simulink model "EMT_ML"  (R2024b)
settings: Solver=ode5  StartTime=0.0  StopTime=200  FixedStep=0.002  RelTol=1e-3
model workspace (MAT data in the model file):
  A = 7.3
  B = 2.71
  C0_shift = 200
  C1_shift = 200
  C2_shift = 200
  Cb = 70
  Cd = 0.6
  EMSInputBus = Simulink.Bus
  EMSInputBus.Alignment = -1
  EMSInputBus.PreserveElementDimensions = 0
  EMSInputBus.Elements_internal(1) = Simulink.BusElement
  EMSInputBus.Elements_internal(1).DimensionsMode = 'Fixed'
  EMSInputBus.Elements_internal(1).SamplingMode = 'Sample based'
  EMSInputBus.Elements_internal(1).SampleTime = -1
  EMSInputBus.Elements_internal(1).Name = 'legacy'
  EMSInputBus.Elements_internal(1).DataType_internal = 'double'
  EMSInputBus.Elements_internal(1).Complexity = 'real'
  EMSInputBus.Elements_internal(1).Dimensions = 19
  EMSInputBus.Elements_internal(2) = Simulink.BusElement
  EMSInputBus.Elements_internal(2).DimensionsMode = 'Fixed'
  EMSInputBus.Elements_internal(2).SamplingMode = 'Sample based'
  EMSInputBus.Elements_internal(2).SampleTime = -1
  EMSInputBus.Elements_internal(2).Name = 'observation'
  EMSInputBus.Elements_internal(2).DataType_internal = 'double'
  EMSInputBus.Elements_internal(2).Complexity = 'real'
  EMSInputBus.Elements_internal(2).Dimensions = 20
  EMSInputBus.Elements_internal(3) = Simulink.BusElement
  EMSInputBus.Elements_internal(3).DimensionsMode = 'Fixed'
  EMSInputBus.Elements_internal(3).SamplingMode = 'Sample based'
  EMSInputBus.Elements_internal(3).SampleTime = -1
  EMSInputBus.Elements_internal(3).Name = 'original_action'
  EMSInputBus.Elements_internal(3).DataType_internal = 'double'
  EMSInputBus.Elements_internal(3).Complexity = 'real'
  EMSInputBus.Elements_internal(3).Dimensions = 4
  EMSInputBus.DataScope = 'Auto'
  Fb_max = 247500
  JA = 0.4
  JB = 0.4
  JZ = 0.4
  Jc1r2 = 0.01
  Jc3r4 = 0.01
  Jc4 = 0.01
  Je = 2.5
  Jh = 0.01
  Jq1 = 0.01
  Jq2 = 0.01
  Jr1 = 0.01
  Jr3s4 = 0.01
  Js123 = 0.01
  L = 4.472
  NE = [1600 1600 1600 1600 1600 1600 1600 1600 1600 1600 1600 1600 ... (840 elements, 30x28)]
  N_Te = 30
  N_ne = 28
  PE = [0 100.366530527 133.710336161 167.221698607 195.706356687 221.845219395 250.497434286 278.144308305 305.288511886 330.086920096 352.87464656 374.489475338 ... (840 elements, 30x28)]
  PN0 = 0
  Pb_epr = [-45 -45 -40 -30 0 30 40 45 45]
  Pb_max = [0 40 45 45 45]
  Pb_min = [-45 -45 -45 -40 0]
  Pe_ass = 230
  Pe_max = 1103
  Peg = [0 100 120 140 160 180 200 220 240 260 280 300 320 340 360 380 400 420 440 460 480 500 520 540 560 580 600 620 640 660 680 700 720 740 760 780 800 820 840 860 880 900 920 940 960 980 1000 1020 1040 1060 1080 1100 1200]
  R_map = [0.09 0.089 0.09 0.091 0.092 0.093 0.094 0.095 0.096 0.097 0.098]
  SF_C0 = 1.5
  SF_C1 = 1.5
  SF_C2 = 1.5
  SF_Z1 = 1.5
  SF_Z2 = 1.5
  SF_ZD = 1.5
  SOC0 = 60
  SOC_epr = [30 31 50 59 60 61 70 79 80]
  SOC_map = [0 10 20 30 40 50 60 70 80 90 100]
  TA_max_map = [588.855 593.803361345 598.83559322 603.953846154 609.160344828 614.457391304 619.847368421 625.332743363 630.916071429 636.6 642.387272727 648.280733945 654.283333333 660.398130841 666.628301887 672.977142857 679.448076923 686.044660194 692.770588235 699.62970297 706.626 713.763636364 721.046938776 728.480412371 736.06875 743.816842105 751.729787234 759.812903226 768.07173913 776.512087912 785.14 793.961797753 802.984090909 812.213793103 821.658139535 831.324705882 841.221428571 851.356626506 861.73902439 872.377777778 883.2825 894.463291139 905.930769231 917.696103896 929.771052632 942.168 954.9 967.980821918 981.425 995.247887324 1009.46571429 1024.09565217 1039.15588235 1054.66567164 1070.64545455 1087.11692308 1110 1110 1110 1087.11692308 1070.64545455 1054.66567164 1039.15588235 1024.09565217 1009.46571429 995.247887324 981.425 967.980821918 954.9 942.168 929.771052632 917.696103896 905.930769231 894.463291139 883.2825 872.377777778 861.73902439 851.356626506 841.221428571 831.324705882 821.658139535 812.213793103 802.984090909 793.961797753 785.14 776.512087912 768.07173913 759.812903226 751.729787234 743.816842105 736.06875 728.480412371 721.046938776 713.763636364 706.626 699.62970297 692.770588235 686.044660194 679.448076923 672.977142857 666.628301887 660.398130841 654.283333333 648.280733945 642.387272727 636.6 630.916071429 625.332743363 619.847368421 614.457391304 609.160344828 603.953846154 598.83559322 593.803361345 588.855]
  TA_min_map = [-588.855 -593.803361345 -598.83559322 -603.953846154 -609.160344828 -614.457391304 -619.847368421 -625.332743363 -630.916071429 -636.6 -642.387272727 -648.280733945 -654.283333333 -660.398130841 -666.628301887 -672.977142857 -679.448076923 -686.044660194 -692.770588235 -699.62970297 -706.626 -713.763636364 -721.046938776 -728.480412371 -736.06875 -743.816842105 -751.729787234 -759.812903226 -768.07173913 -776.512087912 -785.14 -793.961797753 -802.984090909 -812.213793103 -821.658139535 -831.324705882 -841.221428571 -851.356626506 -861.73902439 -872.377777778 -883.2825 -894.463291139 -905.930769231 -917.696103896 -929.771052632 -942.168 -954.9 -967.980821918 -981.425 -995.247887324 -1009.46571429 -1024.09565217 -1039.15588235 -1054.66567164 -1070.64545455 -1087.11692308 -1110 -1110 -1110 -1087.11692308 -1070.64545455 -1054.66567164 -1039.15588235 -1024.09565217 -1009.46571429 -995.247887324 -981.425 -967.980821918 -954.9 -942.168 -929.771052632 -917.696103896 -905.930769231 -894.463291139 -883.2825 -872.377777778 -861.73902439 -851.356626506 -841.221428571 -831.324705882 -821.658139535 -812.213793103 -802.984090909 -793.961797753 -785.14 -776.512087912 -768.07173913 -759.812903226 -751.729787234 -743.816842105 -736.06875 -728.480412371 -721.046938776 -713.763636364 -706.626 -699.62970297 -692.770588235 -686.044660194 -679.448076923 -672.977142857 -666.628301887 -660.398130841 -654.283333333 -648.280733945 -642.387272727 -636.6 -630.916071429 -625.332743363 -619.847368421 -614.457391304 -609.160344828 -603.953846154 -598.83559322 -593.803361345 -588.855]
  TAf = 0
  TB_max_map = [588.855 593.803361345 598.83559322 603.953846154 609.160344828 614.457391304 619.847368421 625.332743363 630.916071429 636.6 642.387272727 648.280733945 654.283333333 660.398130841 666.628301887 672.977142857 679.448076923 686.044660194 692.770588235 699.62970297 706.626 713.763636364 721.046938776 728.480412371 736.06875 743.816842105 751.729787234 759.812903226 768.07173913 776.512087912 785.14 793.961797753 802.984090909 812.213793103 821.658139535 831.324705882 841.221428571 851.356626506 861.73902439 872.377777778 883.2825 894.463291139 905.930769231 917.696103896 929.771052632 942.168 954.9 967.980821918 981.425 995.247887324 1009.46571429 1024.09565217 1039.15588235 1054.66567164 1070.64545455 1087.11692308 1110 1110 1110 1087.11692308 1070.64545455 1054.66567164 1039.15588235 1024.09565217 1009.46571429 995.247887324 981.425 967.980821918 954.9 942.168 929.771052632 917.696103896 905.930769231 894.463291139 883.2825 872.377777778 861.73902439 851.356626506 841.221428571 831.324705882 821.658139535 812.213793103 802.984090909 793.961797753 785.14 776.512087912 768.07173913 759.812903226 751.729787234 743.816842105 736.06875 728.480412371 721.046938776 713.763636364 706.626 699.62970297 692.770588235 686.044660194 679.448076923 672.977142857 666.628301887 660.398130841 654.283333333 648.280733945 642.387272727 636.6 630.916071429 625.332743363 619.847368421 614.457391304 609.160344828 603.953846154 598.83559322 593.803361345 588.855]
  TB_min_map = [-588.855 -593.803361345 -598.83559322 -603.953846154 -609.160344828 -614.457391304 -619.847368421 -625.332743363 -630.916071429 -636.6 -642.387272727 -648.280733945 -654.283333333 -660.398130841 -666.628301887 -672.977142857 -679.448076923 -686.044660194 -692.770588235 -699.62970297 -706.626 -713.763636364 -721.046938776 -728.480412371 -736.06875 -743.816842105 -751.729787234 -759.812903226 -768.07173913 -776.512087912 -785.14 -793.961797753 -802.984090909 -812.213793103 -821.658139535 -831.324705882 -841.221428571 -851.356626506 -861.73902439 -872.377777778 -883.2825 -894.463291139 -905.930769231 -917.696103896 -929.771052632 -942.168 -954.9 -967.980821918 -981.425 -995.247887324 -1009.46571429 -1024.09565217 -1039.15588235 -1054.66567164 -1070.64545455 -1087.11692308 -1110 -1110 -1110 -1087.11692308 -1070.64545455 -1054.66567164 -1039.15588235 -1024.09565217 -1009.46571429 -995.247887324 -981.425 -967.980821918 -954.9 -942.168 -929.771052632 -917.696103896 -905.930769231 -894.463291139 -883.2825 -872.377777778 -861.73902439 -851.356626506 -841.221428571 -831.324705882 -821.658139535 -812.213793103 -802.984090909 -793.961797753 -785.14 -776.512087912 -768.07173913 -759.812903226 -751.729787234 -743.816842105 -736.06875 -728.480412371 -721.046938776 -713.763636364 -706.626 -699.62970297 -692.770588235 -686.044660194 -679.448076923 -672.977142857 -666.628301887 -660.398130841 -654.283333333 -648.280733945 -642.387272727 -636.6 -630.916071429 -625.332743363 -619.847368421 -614.457391304 -609.160344828 -603.953846154 -598.83559322 -593.803361345 -588.855]
  TBf = 0
  TE = [0 599 798 998 1168 1324 1495 1660 1822 1970 2106 2235 ... (840 elements, 30x28)]
  TS_A = 0.2
  TS_B = 0.2
  TS_C0 = 0.2
  TS_C1 = 0.2
  TS_C2 = 0.2
  TS_Z = 0.2
  TS_Z1 = 0.2
  TS_Z2 = 0.2
  TS_ZD = 0.2
  TZ_max_map = [537.13125 540.509433962 543.930379747 547.394904459 550.903846154 554.458064516 558.058441558 561.705882353 565.401315789 569.145695364 572.94 576.785234899 580.682432432 584.632653061 588.636986301 592.696551724 596.8125 600.986013986 605.218309859 609.510638298 613.864285714 618.28057554 622.760869565 627.306569343 631.919117647 636.6 641.350746269 646.172932331 651.068181818 656.038167939 661.084615385 666.209302326 671.4140625 676.700787402 682.071428571 687.528 693.072580645 698.707317073 704.43442623 710.256198347 716.175 722.193277311 728.313559322 734.538461538 740.870689655 747.313043478 753.868421053 760.539823009 767.330357143 774.243243243 781.281818182 788.449541284 795.75 803.186915888 810.764150943 818.485714286 826.355769231 834.378640777 842.558823529 850.900990099 859.41 868.090909091 876.948979592 885.989690722 1000 1000 1000 885.989690722 876.948979592 868.090909091 859.41 850.900990099 842.558823529 834.378640777 826.355769231 818.485714286 810.764150943 803.186915888 795.75 788.449541284 781.281818182 774.243243243 767.330357143 760.539823009 753.868421053 747.313043478 740.870689655 734.538461538 728.313559322 722.193277311 716.175 710.256198347 704.43442623 698.707317073 693.072580645 687.528 682.071428571 676.700787402 671.4140625 666.209302326 661.084615385 656.038167939 651.068181818 646.172932331 641.350746269 636.6 631.919117647 627.306569343 622.760869565 618.28057554 613.864285714 609.510638298 605.218309859 600.986013986 596.8125 592.696551724 588.636986301 584.632653061 580.682432432 576.785234899 572.94 569.145695364 565.401315789 561.705882353 558.058441558 554.458064516 550.903846154 547.394904459 543.930379747 540.509433962 537.13125]
  TZ_min_map = [-537.13125 -540.509433962 -543.930379747 -547.394904459 -550.903846154 -554.458064516 -558.058441558 -561.705882353 -565.401315789 -569.145695364 -572.94 -576.785234899 -580.682432432 -584.632653061 -588.636986301 -592.696551724 -596.8125 -600.986013986 -605.218309859 -609.510638298 -613.864285714 -618.28057554 -622.760869565 -627.306569343 -631.919117647 -636.6 -641.350746269 -646.172932331 -651.068181818 -656.038167939 -661.084615385 -666.209302326 -671.4140625 -676.700787402 -682.071428571 -687.528 -693.072580645 -698.707317073 -704.43442623 -710.256198347 -716.175 -722.193277311 -728.313559322 -734.538461538 -740.870689655 -747.313043478 -753.868421053 -760.539823009 -767.330357143 -774.243243243 -781.281818182 -788.449541284 -795.75 -803.186915888 -810.764150943 -818.485714286 -826.355769231 -834.378640777 -842.558823529 -850.900990099 -859.41 -868.090909091 -876.948979592 -885.989690722 -1000 -1000 -1000 -885.989690722 -876.948979592 -868.090909091 -859.41 -850.900990099 -842.558823529 -834.378640777 -826.355769231 -818.485714286 -810.764150943 -803.186915888 -795.75 -788.449541284 -781.281818182 -774.243243243 -767.330357143 -760.539823009 -753.868421053 -747.313043478 -740.870689655 -734.538461538 -728.313559322 -722.193277311 -716.175 -710.256198347 -704.43442623 -698.707317073 -693.072580645 -687.528 -682.071428571 -676.700787402 -671.4140625 -666.209302326 -661.084615385 -656.038167939 -651.068181818 -646.172932331 -641.350746269 -636.6 -631.919117647 -627.306569343 -622.760869565 -618.28057554 -613.864285714 -609.510638298 -605.218309859 -600.986013986 -596.8125 -592.696551724 -588.636986301 -584.632653061 -580.682432432 -576.785234899 -572.94 -569.145695364 -565.401315789 -561.705882353 -558.058441558 -554.458064516 -550.903846154 -547.394904459 -543.930379747 -540.509433962 -537.13125]
  TZf = 0
  T_generator = [0 185 493.333333333 801.666666667 1110 1418.33333333 1726.66666667]
  T_motor = [0 185 493.333333333 801.666666667 1110 1418.33333333 1726.66666667]
  Te_map = [0 599 798 998 1168 1324 1495 1660 1822 1970 2106 2235 2355 2458 2508 2543 2565 2606 2613 2649 2658 2689 2701 2707 2719 2724 2728 2740 2743 2754]
  Te_max = 2754
  Te_max_map = [1168 1324 1495 1660 1822 1970 2106 2235 2355 2458 2543 2606 2658 2701 2728 2743 2754 2743 2740 2724 2719 2707 2689 2649 2613 2565 2508 998]
  Te_start = 1600
  Tef = 100
  Teg = [0 596.8125 636.6 718.741935484 799.916230366 859.41 954.422788606 954.9 996.417391304 1078.98305085 1114.05 1169.26530612 1170.75862069 1243.45461509 1316.0949464 1388.67967853 1414.66666667 1484.85005553 1554.98149519 1608.98901099 1642.83870968 1657.8125 1712.23448276 1777.47673216 1842.67401792 1907.8263865 1790.4375 1849.54076851 1908.60712055 1967.6365907 2026.62921348 2085.5850234 2144.5040549 2203.38634238 2199.16363636 2256.35262042 2313.50696548 2365.61329305 2394.3761194 2422.46017699 2457.05263158 2455.45714286 2509.3059126 2425.96216216 2476.90894353 2527.82820097 2539.62765957 2589.7314544 2606.5511811 2421.51674641 2455.45714286 2500.92857143 2728.28571429]
  Temax = 998
  Time = [0 0.1 0.2 0.3 0.4 0.5 0.6 0.7 0.8 0.9 1 1.1 ... (2001 elements, 1x2001)]
  Time_ele = [0 4 8 12 16 20 24 28 32 36 40 44 48 52 56 60 64 68 72 76 80 84 88 92 96 100 104 108 112 116 120 124 128 132 136 140 144 148 152 156 160 164 168 172 176 180 184 188 192 196 200 204 208 212 216 220 224 228 232 236 240 244 248 252 256 260 264 268 272 276 280 284 288 292 296 300 304 308 312 316 320 324 328 332 336 340 344 348 352 356 360 364 368 372 376 380 384 388 392 396 400 404 408 412 416 420 424 428 432 436 440 444 448 452 456 460 464 468 472 476 480 484 488 492 496 500 504 508 512 516 520 524 528 532 536 540 544 548 552 556 560 564 568 572 576 580 584 588 592 596 600 604 608 612 616 620 624 628 632 636 640 644 648 652 656 660 664 668 672 676 680 684 688 692 696 700 704 708 712 716 720 724 728 732 736 740 744 748 752 756 760 764 768 772 776 780 784 788 792 796 800 804 808 812 816 820 824 828 832 836 840 844 848 852 856 860 864 868 872 876 880 884 888 892 896 900 904 908 912 916 920 924 928 932 936 940 944 948 952 956 960 964 968 972 976 980 984 988 992 996 1000 1004 1008 1012 1016 1020 1024 1028 1032 1036 1040 1044 1048 1052 1056 1060 1064 1068 1072 1076 1080 1084 1088 1092 1096 1100 1104 1108 1112 1116 1120 1124 1128 1132 1136 1140 1144 1148 1152 1156 1160 1164 1168 1172 1176 1180 1184 1188 1192 1196 1200 1204 1208 1212 1216 1220 1224 1228 1232 1236 1240 1244 1248 1252 1256 1260 1264 1268 1272 1276 1280 1284 1288 1292 1296 1300 1304 1308 1312 1316 1320 1324 1328 1332 1336 1340 1344 1348 1352 1356 1360 1364 1368 1372 1376 1380 1384 1388 1392 1396 1400 1404 1408 1412 1416 1420 1424 1428 1432 1436 1440 1444 1448 1452 1456 1460 1464 1468 1472 1476 1480 1484 1488 1492 1496 1500 1504 1508 1512 1516 1520 1524 1528 1532 1536 1540 1544 1548 1552 1556 1560 1564 1568 1572 1576 1580 1584 1588 1592 1596 1600]
  Time_fg = [0 2 4 6 8 10 12 14 16 18 20 22 ... (801 elements, 1x801)]
  Tmax_C0 = 2754
  Tmax_C1 = 3505.25455609
  Tmax_C2 = 3505.25455609
  Tmax_Z1 = 5584.80955498
  Tmax_Z2 = 16307.6439005
  Tmax_ZD = 3855.6
  Ts_e = 0.1
  Uoc_map = [814.5 917 933.25 945.75 958.25 969.25 978 985.25 993.25 1003.25 1050]
  V_Shift12 = 32
  V_Shift21 = 25
  V_Start = 10
  Voltage0 = 900
  Voltage_epr = [750 760 900 1000 1050]
  Y_engine = 0.955
  Yc = 0.98
  Yh = 0.96
  Yo = 0.92
  Yq = 0.94
  Z1_shift = 200
  Z2_shift = 200
  a11 = 1.54241568346
  a11_L = 1.54241568346
  a12 = -3.86074191629
  a12_L = 2.43173643789
  a21 = -1.04963112005
  a22 = 2.46948356808
  b11 = 0
  b11_L = 0
  b12 = 3.33
  b12_L = 7.8036
  b21 = 2.23571428571
  b22 = -2.13
  c11 = -0.648333656565
  c12 = 0
  c21 = -0.648333656565
  c22 = 0.680511182109
  controller_id = 1
  controller_name = 'Existing heuristic-grid EMS'
  cycle_grade = [0 0 0 0 0 0 0 0 0 0 0 0 ... (2001 elements, 1x2001)]
  cycle_road = [0.045 0.045 0.045 0.045 0.045 0.045 0.045 0.045 0.045 0.045 0.045 0.045 ... (2001 elements, 1x2001)]
  cycle_steering = [0 0 0 0 0 0 0 0 0 0 0 0 ... (2001 elements, 1x2001)]
  cycle_time = [0 0.1 0.2 0.3 0.4 0.5 0.6 0.7 0.8 0.9 1 1.1 ... (2001 elements, 1x2001)]
  d11 = -0.751666343435
  d12 = 0.3003003003
  d21 = -0.751666343435
  d22 = 0.319488817891
  e11 = -1.54241568346
  e12 = 0
  e21 = 1.04963112005
  e22 = -2.23571428571
  eff_generator = [0.8  0.8  0.84  0.84  0.83  0.85  0.83  0.83  0.83  0.8  0.8  0.8; 0.8  0.85  0.92  0.92  0.95  0.88  0.88  0.89  0.92  0.92  0.9  0.92; 0.79  0.88  0.95  0.95  0.95  0.96  0.95  0.92  0.9  0.95  0.8  0.8; 0.79  0.85  0.95  0.95  0.96  0.95  0.95  0.9  0.85  0.75  0.75  0.75; 0.76  0.8  0.9  0.92  0.94  0.9  0.75  0.75  0.75  0.75  0.75  0.75; 0.74  0.79  0.85  0.9  0.91  0.75  0.75  0.75  0.75  0.75  0.75  0.75; 0.72  0.76  0.8  0.83  0.75  0.75  0.75  0.75  0.75  0.75  0.75  0.75]
  eff_motor = [0.8  0.8  0.84  0.84  0.83  0.85  0.83  0.83  0.83  0.8  0.8  0.8; 0.8  0.85  0.92  0.92  0.95  0.88  0.88  0.89  0.92  0.92  0.9  0.92; 0.79  0.88  0.95  0.95  0.95  0.96  0.95  0.92  0.9  0.95  0.8  0.8; 0.79  0.85  0.95  0.95  0.96  0.95  0.95  0.9  0.85  0.75  0.75  0.75; 0.76  0.8  0.9  0.92  0.94  0.9  0.75  0.75  0.75  0.75  0.75  0.75; 0.74  0.79  0.85  0.9  0.91  0.75  0.75  0.75  0.75  0.75  0.75  0.75; 0.72  0.76  0.8  0.83  0.75  0.75  0.75  0.75  0.75  0.75  0.75  0.75]
  ele_map = [10 11.46 14.13 19.24 20.94 23.21 20.29 20.23 22.28 17.66 16.24 18.95 ... (401 elements, 1x401)]
  ems_runtime_config.paths.root = 'C:\Users\LAPTOP1210\Desktop\张东好(hun)\Optimal1103_for_Matlab2015b(好哥毕业模型程序无问题)\ml_ems'
  ems_runtime_config.paths.project = 'C:\Users\LAPTOP1210\Desktop\张东好(hun)\Optimal1103_for_Matlab2015b(好哥毕业模型程序无问题)'
  ems_runtime_config.paths.results = 'C:\Users\LAPTOP1210\Desktop\张东好(hun)\Optimal1103_for_Matlab2015b(好哥毕业模型程序无问题)\ml_ems\results'
  ems_runtime_config.paths.datasets = 'C:\Users\LAPTOP1210\Desktop\张东好(hun)\Optimal1103_for_Matlab2015b(好哥毕业模型程序无问题)\ml_ems\datasets'
  ems_runtime_config.paths.models = 'C:\Users\LAPTOP1210\Desktop\张东好(hun)\Optimal1103_for_Matlab2015b(好哥毕业模型程序无问题)\ml_ems\models'
  ems_runtime_config.p.A = 7.3
  ems_runtime_config.p.B = 2.71
  ems_runtime_config.p.C0_shift = 200
  ems_runtime_config.p.C1_shift = 200
  ems_runtime_config.p.C2_shift = 200
  ems_runtime_config.p.Cb = 70
  ems_runtime_config.p.Cd = 0.6
  ems_runtime_config.p.Fb_max = 247500
  ems_runtime_config.p.JA = 0.4
  ems_runtime_config.p.JB = 0.4
  ems_runtime_config.p.JZ = 0.4
  ems_runtime_config.p.Jc1r2 = 0.01
  ems_runtime_config.p.Jc3r4 = 0.01
  ems_runtime_config.p.Jc4 = 0.01
  ems_runtime_config.p.Je = 2.5
  ems_runtime_config.p.Jh = 0.01
  ems_runtime_config.p.Jq1 = 0.01
  ems_runtime_config.p.Jq2 = 0.01
  ems_runtime_config.p.Jr1 = 0.01
  ems_runtime_config.p.Jr3s4 = 0.01
  ems_runtime_config.p.Js123 = 0.01
  ems_runtime_config.p.L = 4.472
  ems_runtime_config.p.NE = [1600 1600 1600 1600 1600 1600 1600 1600 1600 1600 1600 1600 ... (840 elements, 30x28)]
  ems_runtime_config.p.N_Te = 30
  ems_runtime_config.p.N_ne = 28
  ems_runtime_config.p.PE = [0 100.366530527 133.710336161 167.221698607 195.706356687 221.845219395 250.497434286 278.144308305 305.288511886 330.086920096 352.87464656 374.489475338 ... (840 elements, 30x28)]
  ems_runtime_config.p.PN0 = 0
  ems_runtime_config.p.Pb_epr = [-45 -45 -40 -30 0 30 40 45 45]
  ems_runtime_config.p.Pb_max = [0 40 45 45 45]
  ems_runtime_config.p.Pb_min = [-45 -45 -45 -40 0]
  ems_runtime_config.p.Pe_ass = 230
  ems_runtime_config.p.Pe_max = 1103
  ems_runtime_config.p.Peg = [0 100 120 140 160 180 200 220 240 260 280 300 320 340 360 380 400 420 440 460 480 500 520 540 560 580 600 620 640 660 680 700 720 740 760 780 800 820 840 860 880 900 920 940 960 980 1000 1020 1040 1060 1080 1100 1200]
  ems_runtime_config.p.R_map = [0.09 0.089 0.09 0.091 0.092 0.093 0.094 0.095 0.096 0.097 0.098]
  ems_runtime_config.p.SF_C0 = 1.5
  ems_runtime_config.p.SF_C1 = 1.5
  ems_runtime_config.p.SF_C2 = 1.5
  ems_runtime_config.p.SF_Z1 = 1.5
  ems_runtime_config.p.SF_Z2 = 1.5
  ems_runtime_config.p.SF_ZD = 1.5
  ems_runtime_config.p.SOC0 = 60
  ems_runtime_config.p.SOC_epr = [30 31 50 59 60 61 70 79 80]
  ems_runtime_config.p.SOC_map = [0 10 20 30 40 50 60 70 80 90 100]
  ems_runtime_config.p.TA_max_map = [588.855 593.803361345 598.83559322 603.953846154 609.160344828 614.457391304 619.847368421 625.332743363 630.916071429 636.6 642.387272727 648.280733945 654.283333333 660.398130841 666.628301887 672.977142857 679.448076923 686.044660194 692.770588235 699.62970297 706.626 713.763636364 721.046938776 728.480412371 736.06875 743.816842105 751.729787234 759.812903226 768.07173913 776.512087912 785.14 793.961797753 802.984090909 812.213793103 821.658139535 831.324705882 841.221428571 851.356626506 861.73902439 872.377777778 883.2825 894.463291139 905.930769231 917.696103896 929.771052632 942.168 954.9 967.980821918 981.425 995.247887324 1009.46571429 1024.09565217 1039.15588235 1054.66567164 1070.64545455 1087.11692308 1110 1110 1110 1087.11692308 1070.64545455 1054.66567164 1039.15588235 1024.09565217 1009.46571429 995.247887324 981.425 967.980821918 954.9 942.168 929.771052632 917.696103896 905.930769231 894.463291139 883.2825 872.377777778 861.73902439 851.356626506 841.221428571 831.324705882 821.658139535 812.213793103 802.984090909 793.961797753 785.14 776.512087912 768.07173913 759.812903226 751.729787234 743.816842105 736.06875 728.480412371 721.046938776 713.763636364 706.626 699.62970297 692.770588235 686.044660194 679.448076923 672.977142857 666.628301887 660.398130841 654.283333333 648.280733945 642.387272727 636.6 630.916071429 625.332743363 619.847368421 614.457391304 609.160344828 603.953846154 598.83559322 593.803361345 588.855]
  ems_runtime_config.p.TA_min_map = [-588.855 -593.803361345 -598.83559322 -603.953846154 -609.160344828 -614.457391304 -619.847368421 -625.332743363 -630.916071429 -636.6 -642.387272727 -648.280733945 -654.283333333 -660.398130841 -666.628301887 -672.977142857 -679.448076923 -686.044660194 -692.770588235 -699.62970297 -706.626 -713.763636364 -721.046938776 -728.480412371 -736.06875 -743.816842105 -751.729787234 -759.812903226 -768.07173913 -776.512087912 -785.14 -793.961797753 -802.984090909 -812.213793103 -821.658139535 -831.324705882 -841.221428571 -851.356626506 -861.73902439 -872.377777778 -883.2825 -894.463291139 -905.930769231 -917.696103896 -929.771052632 -942.168 -954.9 -967.980821918 -981.425 -995.247887324 -1009.46571429 -1024.09565217 -1039.15588235 -1054.66567164 -1070.64545455 -1087.11692308 -1110 -1110 -1110 -1087.11692308 -1070.64545455 -1054.66567164 -1039.15588235 -1024.09565217 -1009.46571429 -995.247887324 -981.425 -967.980821918 -954.9 -942.168 -929.771052632 -917.696103896 -905.930769231 -894.463291139 -883.2825 -872.377777778 -861.73902439 -851.356626506 -841.221428571 -831.324705882 -821.658139535 -812.213793103 -802.984090909 -793.961797753 -785.14 -776.512087912 -768.07173913 -759.812903226 -751.729787234 -743.816842105 -736.06875 -728.480412371 -721.046938776 -713.763636364 -706.626 -699.62970297 -692.770588235 -686.044660194 -679.448076923 -672.977142857 -666.628301887 -660.398130841 -654.283333333 -648.280733945 -642.387272727 -636.6 -630.916071429 -625.332743363 -619.847368421 -614.457391304 -609.160344828 -603.953846154 -598.83559322 -593.803361345 -588.855]
  ems_runtime_config.p.TAf = 0
  ems_runtime_config.p.TB_max_map = [588.855 593.803361345 598.83559322 603.953846154 609.160344828 614.457391304 619.847368421 625.332743363 630.916071429 636.6 642.387272727 648.280733945 654.283333333 660.398130841 666.628301887 672.977142857 679.448076923 686.044660194 692.770588235 699.62970297 706.626 713.763636364 721.046938776 728.480412371 736.06875 743.816842105 751.729787234 759.812903226 768.07173913 776.512087912 785.14 793.961797753 802.984090909 812.213793103 821.658139535 831.324705882 841.221428571 851.356626506 861.73902439 872.377777778 883.2825 894.463291139 905.930769231 917.696103896 929.771052632 942.168 954.9 967.980821918 981.425 995.247887324 1009.46571429 1024.09565217 1039.15588235 1054.66567164 1070.64545455 1087.11692308 1110 1110 1110 1087.11692308 1070.64545455 1054.66567164 1039.15588235 1024.09565217 1009.46571429 995.247887324 981.425 967.980821918 954.9 942.168 929.771052632 917.696103896 905.930769231 894.463291139 883.2825 872.377777778 861.73902439 851.356626506 841.221428571 831.324705882 821.658139535 812.213793103 802.984090909 793.961797753 785.14 776.512087912 768.07173913 759.812903226 751.729787234 743.816842105 736.06875 728.480412371 721.046938776 713.763636364 706.626 699.62970297 692.770588235 686.044660194 679.448076923 672.977142857 666.628301887 660.398130841 654.283333333 648.280733945 642.387272727 636.6 630.916071429 625.332743363 619.847368421 614.457391304 609.160344828 603.953846154 598.83559322 593.803361345 588.855]
  ems_runtime_config.p.TB_min_map = [-588.855 -593.803361345 -598.83559322 -603.953846154 -609.160344828 -614.457391304 -619.847368421 -625.332743363 -630.916071429 -636.6 -642.387272727 -648.280733945 -654.283333333 -660.398130841 -666.628301887 -672.977142857 -679.448076923 -686.044660194 -692.770588235 -699.62970297 -706.626 -713.763636364 -721.046938776 -728.480412371 -736.06875 -743.816842105 -751.729787234 -759.812903226 -768.07173913 -776.512087912 -785.14 -793.961797753 -802.984090909 -812.213793103 -821.658139535 -831.324705882 -841.221428571 -851.356626506 -861.73902439 -872.377777778 -883.2825 -894.463291139 -905.930769231 -917.696103896 -929.771052632 -942.168 -954.9 -967.980821918 -981.425 -995.247887324 -1009.46571429 -1024.09565217 -1039.15588235 -1054.66567164 -1070.64545455 -1087.11692308 -1110 -1110 -1110 -1087.11692308 -1070.64545455 -1054.66567164 -1039.15588235 -1024.09565217 -1009.46571429 -995.247887324 -981.425 -967.980821918 -954.9 -942.168 -929.771052632 -917.696103896 -905.930769231 -894.463291139 -883.2825 -872.377777778 -861.73902439 -851.356626506 -841.221428571 -831.324705882 -821.658139535 -812.213793103 -802.984090909 -793.961797753 -785.14 -776.512087912 -768.07173913 -759.812903226 -751.729787234 -743.816842105 -736.06875 -728.480412371 -721.046938776 -713.763636364 -706.626 -699.62970297 -692.770588235 -686.044660194 -679.448076923 -672.977142857 -666.628301887 -660.398130841 -654.283333333 -648.280733945 -642.387272727 -636.6 -630.916071429 -625.332743363 -619.847368421 -614.457391304 -609.160344828 -603.953846154 -598.83559322 -593.803361345 -588.855]
  ems_runtime_config.p.TBf = 0
  ems_runtime_config.p.TE = [0 599 798 998 1168 1324 1495 1660 1822 1970 2106 2235 ... (840 elements, 30x28)]
  ems_runtime_config.p.TS_A = 0.2
  ems_runtime_config.p.TS_B = 0.2
  ems_runtime_config.p.TS_C0 = 0.2
  ems_runtime_config.p.TS_C1 = 0.2
  ems_runtime_config.p.TS_C2 = 0.2
  ems_runtime_config.p.TS_Z = 0.2
  ems_runtime_config.p.TS_Z1 = 0.2
  ems_runtime_config.p.TS_Z2 = 0.2
  ems_runtime_config.p.TS_ZD = 0.2
  ems_runtime_config.p.TZ_max_map = [537.13125 540.509433962 543.930379747 547.394904459 550.903846154 554.458064516 558.058441558 561.705882353 565.401315789 569.145695364 572.94 576.785234899 580.682432432 584.632653061 588.636986301 592.696551724 596.8125 600.986013986 605.218309859 609.510638298 613.864285714 618.28057554 622.760869565 627.306569343 631.919117647 636.6 641.350746269 646.172932331 651.068181818 656.038167939 661.084615385 666.209302326 671.4140625 676.700787402 682.071428571 687.528 693.072580645 698.707317073 704.43442623 710.256198347 716.175 722.193277311 728.313559322 734.538461538 740.870689655 747.313043478 753.868421053 760.539823009 767.330357143 774.243243243 781.281818182 788.449541284 795.75 803.186915888 810.764150943 818.485714286 826.355769231 834.378640777 842.558823529 850.900990099 859.41 868.090909091 876.948979592 885.989690722 1000 1000 1000 885.989690722 876.948979592 868.090909091 859.41 850.900990099 842.558823529 834.378640777 826.355769231 818.485714286 810.764150943 803.186915888 795.75 788.449541284 781.281818182 774.243243243 767.330357143 760.539823009 753.868421053 747.313043478 740.870689655 734.538461538 728.313559322 722.193277311 716.175 710.256198347 704.43442623 698.707317073 693.072580645 687.528 682.071428571 676.700787402 671.4140625 666.209302326 661.084615385 656.038167939 651.068181818 646.172932331 641.350746269 636.6 631.919117647 627.306569343 622.760869565 618.28057554 613.864285714 609.510638298 605.218309859 600.986013986 596.8125 592.696551724 588.636986301 584.632653061 580.682432432 576.785234899 572.94 569.145695364 565.401315789 561.705882353 558.058441558 554.458064516 550.903846154 547.394904459 543.930379747 540.509433962 537.13125]
  ems_runtime_config.p.TZ_min_map = [-537.13125 -540.509433962 -543.930379747 -547.394904459 -550.903846154 -554.458064516 -558.058441558 -561.705882353 -565.401315789 -569.145695364 -572.94 -576.785234899 -580.682432432 -584.632653061 -588.636986301 -592.696551724 -596.8125 -600.986013986 -605.218309859 -609.510638298 -613.864285714 -618.28057554 -622.760869565 -627.306569343 -631.919117647 -636.6 -641.350746269 -646.172932331 -651.068181818 -656.038167939 -661.084615385 -666.209302326 -671.4140625 -676.700787402 -682.071428571 -687.528 -693.072580645 -698.707317073 -704.43442623 -710.256198347 -716.175 -722.193277311 -728.313559322 -734.538461538 -740.870689655 -747.313043478 -753.868421053 -760.539823009 -767.330357143 -774.243243243 -781.281818182 -788.449541284 -795.75 -803.186915888 -810.764150943 -818.485714286 -826.355769231 -834.378640777 -842.558823529 -850.900990099 -859.41 -868.090909091 -876.948979592 -885.989690722 -1000 -1000 -1000 -885.989690722 -876.948979592 -868.090909091 -859.41 -850.900990099 -842.558823529 -834.378640777 -826.355769231 -818.485714286 -810.764150943 -803.186915888 -795.75 -788.449541284 -781.281818182 -774.243243243 -767.330357143 -760.539823009 -753.868421053 -747.313043478 -740.870689655 -734.538461538 -728.313559322 -722.193277311 -716.175 -710.256198347 -704.43442623 -698.707317073 -693.072580645 -687.528 -682.071428571 -676.700787402 -671.4140625 -666.209302326 -661.084615385 -656.038167939 -651.068181818 -646.172932331 -641.350746269 -636.6 -631.919117647 -627.306569343 -622.760869565 -618.28057554 -613.864285714 -609.510638298 -605.218309859 -600.986013986 -596.8125 -592.696551724 -588.636986301 -584.632653061 -580.682432432 -576.785234899 -572.94 -569.145695364 -565.401315789 -561.705882353 -558.058441558 -554.458064516 -550.903846154 -547.394904459 -543.930379747 -540.509433962 -537.13125]
  ems_runtime_config.p.TZf = 0
  ems_runtime_config.p.T_generator = [0 185 493.333333333 801.666666667 1110 1418.33333333 1726.66666667]
  ems_runtime_config.p.T_motor = [0 185 493.333333333 801.666666667 1110 1418.33333333 1726.66666667]
  ems_runtime_config.p.Te_map = [0 599 798 998 1168 1324 1495 1660 1822 1970 2106 2235 2355 2458 2508 2543 2565 2606 2613 2649 2658 2689 2701 2707 2719 2724 2728 2740 2743 2754]
  ems_runtime_config.p.Te_max = 2754
  ems_runtime_config.p.Te_max_map = [1168 1324 1495 1660 1822 1970 2106 2235 2355 2458 2543 2606 2658 2701 2728 2743 2754 2743 2740 2724 2719 2707 2689 2649 2613 2565 2508 998]
  ems_runtime_config.p.Te_start = 1600
  ems_runtime_config.p.Tef = 100
  ems_runtime_config.p.Teg = [0 596.8125 636.6 718.741935484 799.916230366 859.41 954.422788606 954.9 996.417391304 1078.98305085 1114.05 1169.26530612 1170.75862069 1243.45461509 1316.0949464 1388.67967853 1414.66666667 1484.85005553 1554.98149519 1608.98901099 1642.83870968 1657.8125 1712.23448276 1777.47673216 1842.67401792 1907.8263865 1790.4375 1849.54076851 1908.60712055 1967.6365907 2026.62921348 2085.5850234 2144.5040549 2203.38634238 2199.16363636 2256.35262042 2313.50696548 2365.61329305 2394.3761194 2422.46017699 2457.05263158 2455.45714286 2509.3059126 2425.96216216 2476.90894353 2527.82820097 2539.62765957 2589.7314544 2606.5511811 2421.51674641 2455.45714286 2500.92857143 2728.28571429]
  ems_runtime_config.p.Temax = 998
  ems_runtime_config.p.Tmax_C0 = 2754
  ems_runtime_config.p.Tmax_C1 = 3505.25455609
  ems_runtime_config.p.Tmax_C2 = 3505.25455609
  ems_runtime_config.p.Tmax_Z1 = 5584.80955498
  ems_runtime_config.p.Tmax_Z2 = 16307.6439005
  ems_runtime_config.p.Tmax_ZD = 3855.6
  ems_runtime_config.p.Ts_e = 0.1
  ems_runtime_config.p.Uoc_map = [814.5 917 933.25 945.75 958.25 969.25 978 985.25 993.25 1003.25 1050]
  ems_runtime_config.p.V_Shift12 = 32
  ems_runtime_config.p.V_Shift21 = 25
  ems_runtime_config.p.V_Start = 10
  ems_runtime_config.p.Voltage0 = 900
  ems_runtime_config.p.Voltage_epr = [750 760 900 1000 1050]
  ems_runtime_config.p.Y_engine = 0.955
  ems_runtime_config.p.Yc = 0.98
  ems_runtime_config.p.Yh = 0.96
  ems_runtime_config.p.Yo = 0.92
  ems_runtime_config.p.Yq = 0.94
  ems_runtime_config.p.Z1_shift = 200
  ems_runtime_config.p.Z2_shift = 200
  ems_runtime_config.p.a11 = 1.54241568346
  ems_runtime_config.p.a11_L = 1.54241568346
  ems_runtime_config.p.a12 = -3.86074191629
  ems_runtime_config.p.a12_L = 2.43173643789
  ems_runtime_config.p.a21 = -1.04963112005
  ems_runtime_config.p.a22 = 2.46948356808
  ems_runtime_config.p.b11 = 0
  ems_runtime_config.p.b11_L = 0
  ems_runtime_config.p.b12 = 3.33
  ems_runtime_config.p.b12_L = 7.8036
  ems_runtime_config.p.b21 = 2.23571428571
  ems_runtime_config.p.b22 = -2.13
  ems_runtime_config.p.c11 = -0.648333656565
  ems_runtime_config.p.c12 = 0
  ems_runtime_config.p.c21 = -0.648333656565
  ems_runtime_config.p.c22 = 0.680511182109
  ems_runtime_config.p.d11 = -0.751666343435
  ems_runtime_config.p.d12 = 0.3003003003
  ems_runtime_config.p.d21 = -0.751666343435
  ems_runtime_config.p.d22 = 0.319488817891
  ems_runtime_config.p.e11 = -1.54241568346
  ems_runtime_config.p.e12 = 0
  ems_runtime_config.p.e21 = 1.04963112005
  ems_runtime_config.p.e22 = -2.23571428571
  ems_runtime_config.p.eff_generator = [0.8  0.8  0.84  0.84  0.83  0.85  0.83  0.83  0.83  0.8  0.8  0.8; 0.8  0.85  0.92  0.92  0.95  0.88  0.88  0.89  0.92  0.92  0.9  0.92; 0.79  0.88  0.95  0.95  0.95  0.96  0.95  0.92  0.9  0.95  0.8  0.8; 0.79  0.85  0.95  0.95  0.96  0.95  0.95  0.9  0.85  0.75  0.75  0.75; 0.76  0.8  0.9  0.92  0.94  0.9  0.75  0.75  0.75  0.75  0.75  0.75; 0.74  0.79  0.85  0.9  0.91  0.75  0.75  0.75  0.75  0.75  0.75  0.75; 0.72  0.76  0.8  0.83  0.75  0.75  0.75  0.75  0.75  0.75  0.75  0.75]
  ems_runtime_config.p.eff_motor = [0.8  0.8  0.84  0.84  0.83  0.85  0.83  0.83  0.83  0.8  0.8  0.8; 0.8  0.85  0.92  0.92  0.95  0.88  0.88  0.89  0.92  0.92  0.9  0.92; 0.79  0.88  0.95  0.95  0.95  0.96  0.95  0.92  0.9  0.95  0.8  0.8; 0.79  0.85  0.95  0.95  0.96  0.95  0.95  0.9  0.85  0.75  0.75  0.75; 0.76  0.8  0.9  0.92  0.94  0.9  0.75  0.75  0.75  0.75  0.75  0.75; 0.74  0.79  0.85  0.9  0.91  0.75  0.75  0.75  0.75  0.75  0.75  0.75; 0.72  0.76  0.8  0.83  0.75  0.75  0.75  0.75  0.75  0.75  0.75  0.75]
  ems_runtime_config.p.f11 = -3.86074191629
  ems_runtime_config.p.f12 = 3.33
  ems_runtime_config.p.f21 = 2.46948356808
  ems_runtime_config.p.f22 = -2.13
  ems_runtime_config.p.fg = 0.045
  ems_runtime_config.p.fuel_gpkwh = [269.874826377 269.874826377 260.084605263 254.895150301 249.802821062 244.062054381 234.972466555 226.630558735 223.93243551 227.612775381 231.379615385 228.983738255 ... (840 elements, 30x28)]
  ems_runtime_config.p.fuel_map = [269.874826377 269.874826377 260.084605263 254.895150301 249.802821062 244.062054381 234.972466555 226.630558735 223.93243551 227.612775381 231.379615385 228.983738255 ... (840 elements, 30x28)]
  ems_runtime_config.p.fuel_map_N = [269.874826377 269.874826377 260.084605263 254.895150301 249.802821062 NaN NaN NaN NaN NaN NaN NaN ... (840 elements, 30x28)]
  ems_runtime_config.p.i = 28
  ems_runtime_config.p.ic = 4.42
  ems_runtime_config.p.iq = 1.4
  ems_runtime_config.p.it = 4
  ems_runtime_config.p.j = 30
  ems_runtime_config.p.k1 = 2.13
  ems_runtime_config.p.k2 = 2.13
  ems_runtime_config.p.k3 = 2.33
  ems_runtime_config.p.k4 = 1.92
  ems_runtime_config.p.kh = 2.88
  ems_runtime_config.p.kq = 2.17
  ems_runtime_config.p.kt = 1.83
  ems_runtime_config.p.mass = 45000
  ems_runtime_config.p.miu_max = 0.8
  ems_runtime_config.p.nA_map = [-6000 -5950 -5900 -5850 -5800 -5750 -5700 -5650 -5600 -5550 -5500 -5450 -5400 -5350 -5300 -5250 -5200 -5150 -5100 -5050 -5000 -4950 -4900 -4850 -4800 -4750 -4700 -4650 -4600 -4550 -4500 -4450 -4400 -4350 -4300 -4250 -4200 -4150 -4100 -4050 -4000 -3950 -3900 -3850 -3800 -3750 -3700 -3650 -3600 -3550 -3500 -3450 -3400 -3350 -3300 -3250 -3200 0 3200 3250 3300 3350 3400 3450 3500 3550 3600 3650 3700 3750 3800 3850 3900 3950 4000 4050 4100 4150 4200 4250 4300 4350 4400 4450 4500 4550 4600 4650 4700 4750 4800 4850 4900 4950 5000 5050 5100 5150 5200 5250 5300 5350 5400 5450 5500 5550 5600 5650 5700 5750 5800 5850 5900 5950 6000]
  ems_runtime_config.p.nA_max = 6000
  ems_runtime_config.p.nA_min = -6000
  ems_runtime_config.p.nB_map = [-6000 -5950 -5900 -5850 -5800 -5750 -5700 -5650 -5600 -5550 -5500 -5450 -5400 -5350 -5300 -5250 -5200 -5150 -5100 -5050 -5000 -4950 -4900 -4850 -4800 -4750 -4700 -4650 -4600 -4550 -4500 -4450 -4400 -4350 -4300 -4250 -4200 -4150 -4100 -4050 -4000 -3950 -3900 -3850 -3800 -3750 -3700 -3650 -3600 -3550 -3500 -3450 -3400 -3350 -3300 -3250 -3200 0 3200 3250 3300 3350 3400 3450 3500 3550 3600 3650 3700 3750 3800 3850 3900 3950 4000 4050 4100 4150 4200 4250 4300 4350 4400 4450 4500 4550 4600 4650 4700 4750 4800 4850 4900 4950 5000 5050 5100 5150 5200 5250 5300 5350 5400 5450 5500 5550 5600 5650 5700 5750 5800 5850 5900 5950 6000]
  ems_runtime_config.p.nB_max = 6000
  ems_runtime_config.p.nB_min = -6000
  ems_runtime_config.p.nB_start = 0
  ems_runtime_config.p.nZ_map = [-8000 -7950 -7900 -7850 -7800 -7750 -7700 -7650 -7600 -7550 -7500 -7450 -7400 -7350 -7300 -7250 -7200 -7150 -7100 -7050 -7000 -6950 -6900 -6850 -6800 -6750 -6700 -6650 -6600 -6550 -6500 -6450 -6400 -6350 -6300 -6250 -6200 -6150 -6100 -6050 -6000 -5950 -5900 -5850 -5800 -5750 -5700 -5650 -5600 -5550 -5500 -5450 -5400 -5350 -5300 -5250 -5200 -5150 -5100 -5050 -5000 -4950 -4900 -4850 -4800 0 4800 4850 4900 4950 5000 5050 5100 5150 5200 5250 5300 5350 5400 5450 5500 5550 5600 5650 5700 5750 5800 5850 5900 5950 6000 6050 6100 6150 6200 6250 6300 6350 6400 6450 6500 6550 6600 6650 6700 6750 6800 6850 6900 6950 7000 7050 7100 7150 7200 7250 7300 7350 7400 7450 7500 7550 7600 7650 7700 7750 7800 7850 7900 7950 8000]
  ems_runtime_config.p.nZ_max = 8000
  ems_runtime_config.p.nZ_min = -8000
  ems_runtime_config.p.n_generator = [0 318.5 796.25 1274 1751.75 2229.5 2707.25 3185 3662.75 4140.5 4618.25 7007]
  ems_runtime_config.p.n_motor = [0 318.5 796.25 1274 1751.75 2229.5 2707.25 3185 3662.75 4140.5 4618.25 7007]
  ems_runtime_config.p.ne_idl = 3000
  ems_runtime_config.p.ne_map = [1600 1700 1800 1900 2000 2100 2200 2300 2400 2500 2600 2700 2800 2900 3000 3100 3200 3300 3400 3500 3600 3700 3800 3900 4000 4100 4200 4500]
  ems_runtime_config.p.ne_max = 4200
  ems_runtime_config.p.ne_min = 1600
  ems_runtime_config.p.ne_start = 200
  ems_runtime_config.p.neg = [1600 1600 1800 1860 1910 2000 2001 2200 2300 2301 2400 2450 2610 2611 2612 2613 2700 2701 2702 2730 2790 2880 2900 2901 2902 2903 3200 3201 3202 3203 3204 3205 3206 3207 3300 3301 3302 3310 3350 3390 3420 3500 3501 3700 3701 3702 3760 3761 3810 4180 4200 4200 4200]
  ems_runtime_config.p.no_Shift12 = 1589.43589002
  ems_runtime_config.p.no_Shift21 = 1241.74678908
  ems_runtime_config.p.rz = 0.318
  ems_runtime_config.p.voltage_HighA = 1050
  ems_runtime_config.p.voltage_HighB = 1050
  ems_runtime_config.p.voltage_HighZ = 1050
  ems_runtime_config.p.voltage_LowA = 750
  ems_runtime_config.p.voltage_LowB = 750
  ems_runtime_config.p.voltage_LowZ = 750
  ems_runtime_config.p.Time = [0 0.1 0.2 0.3 0.4 0.5 0.6 0.7 0.8 0.9 1 1.1 ... (2001 elements, 1x2001)]
  ems_runtime_config.p.v_cyc = [0 0 0 0 0 0 0 0 0 0 0 0 ... (2001 elements, 1x2001)]
  ems_runtime_config.p.Time_fg = [0 2 4 6 8 10 12 14 16 18 20 22 ... (801 elements, 1x801)]
  ems_runtime_config.p.fg_map = [0.0125 0.0215 0.0332 0.0452 0.0525 0.0589 0.0584 0.0592 0.0621 0.0576 0.055 0.0572 ... (801 elements, 1x801)]
  ems_runtime_config.p.Time_ele = [0 4 8 12 16 20 24 28 32 36 40 44 48 52 56 60 64 68 72 76 80 84 88 92 96 100 104 108 112 116 120 124 128 132 136 140 144 148 152 156 160 164 168 172 176 180 184 188 192 196 200 204 208 212 216 220 224 228 232 236 240 244 248 252 256 260 264 268 272 276 280 284 288 292 296 300 304 308 312 316 320 324 328 332 336 340 344 348 352 356 360 364 368 372 376 380 384 388 392 396 400 404 408 412 416 420 424 428 432 436 440 444 448 452 456 460 464 468 472 476 480 484 488 492 496 500 504 508 512 516 520 524 528 532 536 540 544 548 552 556 560 564 568 572 576 580 584 588 592 596 600 604 608 612 616 620 624 628 632 636 640 644 648 652 656 660 664 668 672 676 680 684 688 692 696 700 704 708 712 716 720 724 728 732 736 740 744 748 752 756 760 764 768 772 776 780 784 788 792 796 800 804 808 812 816 820 824 828 832 836 840 844 848 852 856 860 864 868 872 876 880 884 888 892 896 900 904 908 912 916 920 924 928 932 936 940 944 948 952 956 960 964 968 972 976 980 984 988 992 996 1000 1004 1008 1012 1016 1020 1024 1028 1032 1036 1040 1044 1048 1052 1056 1060 1064 1068 1072 1076 1080 1084 1088 1092 1096 1100 1104 1108 1112 1116 1120 1124 1128 1132 1136 1140 1144 1148 1152 1156 1160 1164 1168 1172 1176 1180 1184 1188 1192 1196 1200 1204 1208 1212 1216 1220 1224 1228 1232 1236 1240 1244 1248 1252 1256 1260 1264 1268 1272 1276 1280 1284 1288 1292 1296 1300 1304 1308 1312 1316 1320 1324 1328 1332 1336 1340 1344 1348 1352 1356 1360 1364 1368 1372 1376 1380 1384 1388 1392 1396 1400 1404 1408 1412 1416 1420 1424 1428 1432 1436 1440 1444 1448 1452 1456 1460 1464 1468 1472 1476 1480 1484 1488 1492 1496 1500 1504 1508 1512 1516 1520 1524 1528 1532 1536 1540 1544 1548 1552 1556 1560 1564 1568 1572 1576 1580 1584 1588 1592 1596 1600]
  ems_runtime_config.p.ele_map = [10 11.46 14.13 19.24 20.94 23.21 20.29 20.23 22.28 17.66 16.24 18.95 ... (401 elements, 1x401)]
  ems_runtime_config.control.Ts = 0.1
  ems_runtime_config.control.legacy_Ts = 0.02
  ems_runtime_config.control.history = 30
  ems_runtime_config.control.horizon = 20
  ems_runtime_config.control.samples = 256
  ems_runtime_config.control.elite_fraction = 0.1
  ems_runtime_config.control.iterations = 3
  ems_runtime_config.control.knots = 5
  ems_runtime_config.control.soc_min = 0.3
  ems_runtime_config.control.soc_max = 0.8
  ems_runtime_config.control.soc_target = 0.6
  ems_runtime_config.control.voltage_min = 750
  ems_runtime_config.control.voltage_max = 1050
  ems_runtime_config.control.current_max = 80
  ems_runtime_config.control.rate = [5000 20000 20000 20000]
  ems_runtime_config.control.torque_balance_tolerance = 150
  ems_runtime_config.control.constraint_tolerance = 1e-06
  ems_runtime_config.control.engine_efficiency = 0.955
  ems_runtime_config.control.motor_efficiency = 0.8
  ems_runtime_config.control.engine_shaft_fraction = 0.799152311877
  ems_runtime_config.control.transmission_efficiency = 0.8648
  ems_runtime_config.control.engine_drag_Nm = 100
  ems_runtime_config.control.weights.fuel = 1
  ems_runtime_config.control.weights.battery = 1
  ems_runtime_config.control.weights.speed = 0.03
  ems_runtime_config.control.weights.terminal_soc = 20000
  ems_runtime_config.control.weights.slew = 0.02
  ems_runtime_config.control.weights.engine_start = 2
  ems_runtime_config.control.weights.mode_switch = 1
  ems_runtime_config.control.weights.constraint = 100000
  ems_runtime_config.control.weights.risk = 0.5
  ems_runtime_config.control.ecms_factor = 2.5
  ems_runtime_config.control.ecms_soc_gain = 15
  ems_runtime_config.control.no_fuel_map = 0
  ems_runtime_config.control.no_terminal_soc = 0
  ems_runtime_config.control.no_history = 0
  ems_runtime_config.control.no_uncertainty = 0
  ems_runtime_config.control.feature_names = {'v_ref', 'traction_power', 'aux_power', 'road_resistance', 'v_act', 'SOC', 'grade', 'pedal'}
  ems_runtime_config.control.target_names = {'v_ref', 'traction_power', 'aux_power', 'road_resistance'}
  ems_runtime_config.version = 'ems-r2024b-v1'
  ems_runtime_config.seed = 1
  ems_runtime_config.seeds = [1 2 3 4 5]
  ems_runtime_config.controller_id = 1
  ems_runtime_config.controller_name = 'Existing heuristic-grid EMS'
  ems_runtime_config.stop_time = 30
  ems_runtime_config.fast_restart = 0
  ems_runtime_config.parallel = 0
  ems_runtime_config.fuel_density_kg_L = 0.84
  ems_runtime_config.LHV_kJ_kg = 42700
  ems_runtime_config.eta_eq = 0.35
  ems_runtime_config.fuel_assumptions = 'LHV=42.7 MJ/kg, eta_eq=.35 are declared study assumptions, not calibrated vehicle measurements.'
  ems_runtime_config.initial_soc_percent = 60
  ems_runtime_config.mass_scale = 1
  ems_runtime_config.cycle_name = 'city200'
  ems_runtime_config.logging_Ts = 0.1
  ems_runtime_config.model = 'EMT_ML'
  ems_runtime_config.max_wall_seconds = 1800
  ems_runtime_config.ensemble_size = 3
  ems_runtime_config.epochs = 30
  ems_runtime_config.batch_size = 128
  ems_runtime_config.model_dir = 'C:\Users\LAPTOP1210\Desktop\张东好(hun)\Optimal1103_for_Matlab2015b(好哥毕业模型程序无问题)\ml_ems\models\trained'
  ems_runtime_config.training_seeds = [101 102 103 104 105 106]
  ems_runtime_config.validation_seeds = [201 202]
  ems_runtime_config.dataset_duration = 60
  ems_runtime_config.dataset_experts = [1 3 2]
  ems_runtime_config.dp_soc_grid = [0.3 0.305 0.31 0.315 0.32 0.325 0.33 0.335 0.34 0.345 0.35 0.355 0.36 0.365 0.37 0.375 0.38 0.385 0.39 0.395 0.4 0.405 0.41 0.415 0.42 0.425 0.43 0.435 0.44 0.445 0.45 0.455 0.46 0.465 0.47 0.475 0.48 0.485 0.49 0.495 0.5 0.505 0.51 0.515 0.52 0.525 0.53 0.535 0.54 0.545 0.55 0.555 0.56 0.565 0.57 0.575 0.58 0.585 0.59 0.595 0.6 0.605 0.61 0.615 0.62 0.625 0.63 0.635 0.64 0.645 0.65 0.655 0.66 0.665 0.67 0.675 0.68 0.685 0.69 0.695 0.7 0.705 0.71 0.715 0.72 0.725 0.73 0.735 0.74 0.745 0.75 0.755 0.76 0.765 0.77 0.775 0.78 0.785 0.79 0.795 0.8]
  ems_runtime_config.dp_power_grid = [-45 -42 -39 -36 -33 -30 -27 -24 -21 -18 -15 -12 -9 -6 -3 0 3 6 9 12 15 18 21 24 27 30 33 36 39 42 45]
  ems_runtime_config.parity.speed = 0.0001
  ems_runtime_config.parity.soc = 1e-05
  ems_runtime_config.parity.power = 0.001
  ems_runtime_config.parity.relative = 1e-06
  f11 = -3.86074191629
  f12 = 3.33
  f21 = 2.46948356808
  f22 = -2.13
  fg = 0.045
  fg_map = [0.0125 0.0215 0.0332 0.0452 0.0525 0.0589 0.0584 0.0592 0.0621 0.0576 0.055 0.0572 ... (801 elements, 1x801)]
  fuel_gpkwh = [269.874826377 269.874826377 260.084605263 254.895150301 249.802821062 244.062054381 234.972466555 226.630558735 223.93243551 227.612775381 231.379615385 228.983738255 ... (840 elements, 30x28)]
  fuel_map = [269.874826377 269.874826377 260.084605263 254.895150301 249.802821062 244.062054381 234.972466555 226.630558735 223.93243551 227.612775381 231.379615385 228.983738255 ... (840 elements, 30x28)]
  fuel_map_N = [269.874826377 269.874826377 260.084605263 254.895150301 249.802821062 nan nan nan nan nan nan nan ... (840 elements, 30x28)]
  i = 28
  ic = 4.42
  iq = 1.4
  it = 4
  j = 30
  k1 = 2.13
  k2 = 2.13
  k3 = 2.33
  k4 = 1.92
  kh = 2.88
  kq = 2.17
  kt = 1.83
  mass = 45000
  miu_max = 0.8
  nA_map = [-6000 -5950 -5900 -5850 -5800 -5750 -5700 -5650 -5600 -5550 -5500 -5450 -5400 -5350 -5300 -5250 -5200 -5150 -5100 -5050 -5000 -4950 -4900 -4850 -4800 -4750 -4700 -4650 -4600 -4550 -4500 -4450 -4400 -4350 -4300 -4250 -4200 -4150 -4100 -4050 -4000 -3950 -3900 -3850 -3800 -3750 -3700 -3650 -3600 -3550 -3500 -3450 -3400 -3350 -3300 -3250 -3200 0 3200 3250 3300 3350 3400 3450 3500 3550 3600 3650 3700 3750 3800 3850 3900 3950 4000 4050 4100 4150 4200 4250 4300 4350 4400 4450 4500 4550 4600 4650 4700 4750 4800 4850 4900 4950 5000 5050 5100 5150 5200 5250 5300 5350 5400 5450 5500 5550 5600 5650 5700 5750 5800 5850 5900 5950 6000]
  nA_max = 6000
  nA_min = -6000
  nB_map = [-6000 -5950 -5900 -5850 -5800 -5750 -5700 -5650 -5600 -5550 -5500 -5450 -5400 -5350 -5300 -5250 -5200 -5150 -5100 -5050 -5000 -4950 -4900 -4850 -4800 -4750 -4700 -4650 -4600 -4550 -4500 -4450 -4400 -4350 -4300 -4250 -4200 -4150 -4100 -4050 -4000 -3950 -3900 -3850 -3800 -3750 -3700 -3650 -3600 -3550 -3500 -3450 -3400 -3350 -3300 -3250 -3200 0 3200 3250 3300 3350 3400 3450 3500 3550 3600 3650 3700 3750 3800 3850 3900 3950 4000 4050 4100 4150 4200 4250 4300 4350 4400 4450 4500 4550 4600 4650 4700 4750 4800 4850 4900 4950 5000 5050 5100 5150 5200 5250 5300 5350 5400 5450 5500 5550 5600 5650 5700 5750 5800 5850 5900 5950 6000]
  nB_max = 6000
  nB_min = -6000
  nB_start = 0
  nZ_map = [-8000 -7950 -7900 -7850 -7800 -7750 -7700 -7650 -7600 -7550 -7500 -7450 -7400 -7350 -7300 -7250 -7200 -7150 -7100 -7050 -7000 -6950 -6900 -6850 -6800 -6750 -6700 -6650 -6600 -6550 -6500 -6450 -6400 -6350 -6300 -6250 -6200 -6150 -6100 -6050 -6000 -5950 -5900 -5850 -5800 -5750 -5700 -5650 -5600 -5550 -5500 -5450 -5400 -5350 -5300 -5250 -5200 -5150 -5100 -5050 -5000 -4950 -4900 -4850 -4800 0 4800 4850 4900 4950 5000 5050 5100 5150 5200 5250 5300 5350 5400 5450 5500 5550 5600 5650 5700 5750 5800 5850 5900 5950 6000 6050 6100 6150 6200 6250 6300 6350 6400 6450 6500 6550 6600 6650 6700 6750 6800 6850 6900 6950 7000 7050 7100 7150 7200 7250 7300 7350 7400 7450 7500 7550 7600 7650 7700 7750 7800 7850 7900 7950 8000]
  nZ_max = 8000
  nZ_min = -8000
  n_generator = [0 318.5 796.25 1274 1751.75 2229.5 2707.25 3185 3662.75 4140.5 4618.25 7007]
  n_motor = [0 318.5 796.25 1274 1751.75 2229.5 2707.25 3185 3662.75 4140.5 4618.25 7007]
  ne_idl = 3000
  ne_map = [1600 1700 1800 1900 2000 2100 2200 2300 2400 2500 2600 2700 2800 2900 3000 3100 3200 3300 3400 3500 3600 3700 3800 3900 4000 4100 4200 4500]
  ne_max = 4200
  ne_min = 1600
  ne_start = 200
  neg = [1600 1600 1800 1860 1910 2000 2001 2200 2300 2301 2400 2450 2610 2611 2612 2613 2700 2701 2702 2730 2790 2880 2900 2901 2902 2903 3200 3201 3202 3203 3204 3205 3206 3207 3300 3301 3302 3310 3350 3390 3420 3500 3501 3700 3701 3702 3760 3761 3810 4180 4200 4200 4200]
  no_Shift12 = 1589.43589002
  no_Shift21 = 1241.74678908
  rz = 0.318
  startup_feedback_delay_s = 0.002
  startup_power_share = 0.5
  startup_speed_regularizer_rpm = 100
  v_cyc = [0 0 0 0 0 0 0 0 0 0 0 0 ... (2001 elements, 1x2001)]
  voltage_HighA = 1050
  voltage_HighB = 1050
  voltage_HighZ = 1050
  voltage_LowA = 750
  voltage_LowB = 750
  voltage_LowZ = 750
undefined symbols (not defined in the file or in its folder): sigbuilder_block
libraries: fl_lib x82, nesl_utility x55, simulink x49, sdl_lib x10, slpidlib x3, simulink_need_slupdate x3, powerlib_extras x1
(part 1 of 7)
settings Model: Creator=admin  LastModifiedBy=LAPTOP1210
settings SolverCC: AlgebraicLoopSolver=LineSearch  AutoInsertRateTranBlk=on
settings DataIOCC: SaveFormat=Array  SignalLoggingName=state_capture_logs
settings OptimizationCC: BlockReduction=off  OptimizeBlockIOStorage=off  BufferReuse=off  GlobalBufferReuse=off  ExpressionFolding=off  ExpressionDepthLimit=2147483647  LocalBlockOutputs=off  InitFltsAndDblsToZero=on  LifeSpan=inf
settings DebuggingCC: AlgebraicLoopMsg=none  UnderspecifiedInitializationDetection=Classic  SolverPrmCheckMsg=warning  MultiTaskRateTransMsg=warning  FcnCallInpInsideContextMsg=warning  UnconnectedInputMsg=warning  UnconnectedOutputMsg=warning  UnconnectedLineMsg=warning  AllowSymbolicDim=off  StateNameClashWarn=warning  SFUnexpectedBacktrackingDiag=warning  SFNoUnconditionalDefaultTransitionDiag=warning  SFExecutionAtInitializationDiag=none  ArithmeticOperatorsInVariantConditions=warning
settings HardwareCC: ProdBitPerPointer=32  ProdBitPerSizeT=32  ProdBitPerPtrDiffT=32  ProdLargestAtomicFloat=None  ProdIntDivRoundTo=Undefined  ProdEndianess=Unspecified  ProdWordSize=32  ProdHWDeviceType=32-bit Generic
settings ModelReferenceCC: EnableRefExpFcnMdlSchedulingChecks=on  PropagateSignalLabelsOutOfModel=off
settings SFSimCC: SimUseLocalCustomCode=off  CustomCodeUndefinedFunction=UseInterfaceOnly
settings RTWCC: RTWUseLocalCustomCode=off  GPUComputeCapability=3.5
settings CodeAppCC: StateflowObjectComments=on
settings GRTTargetCC: TargetLangStandard=C89/C90 (ANSI)  CombineOutputUpdateFcns=off  GRTInterface=on
settings ConfigComp: CovMetricSettings=dw  CovSaveCumulativeToWorkspaceVar=on  CovSaveSingleToWorkspaceVar=on  CovExternalEMLEnable=off
settings SimscapeCC: ExplicitSolverDiagnosticOptions=none  SimscapeNormalizeSystem=off  SimscapeLogType=all  SimscapeLogName=state_capture_simlog  SimscapeLogLimitData=off

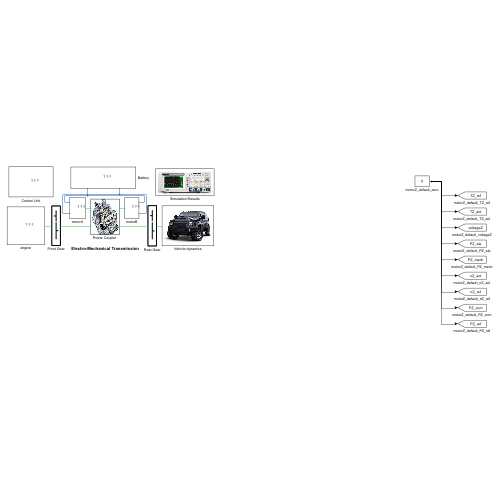
[thumbnail: Simulink's stored preview of the top-level diagram]
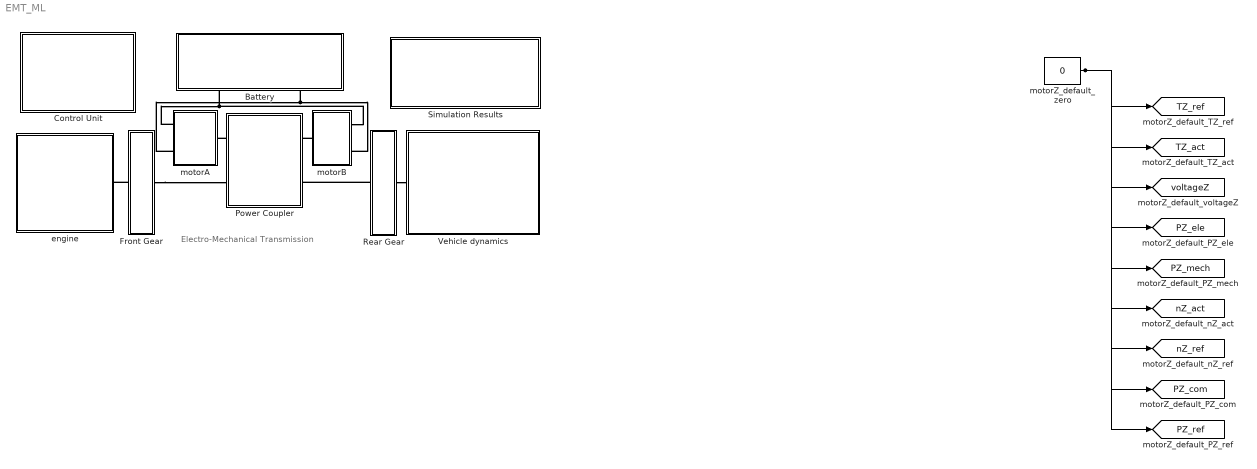
== system EMT_ML ==
  note: Electro-Mechanical Transmission
  Battery : Subsystem
      mask Display: image(imread('power_HEV_powertrain_battery.jpg'))
  Control Unit : Subsystem  SystemSampleTime=0.02
      mask Display: image(imread('power_aircraft_distribution_GCU.jpg','jpg'))
  Front Gear : Subsystem
      mask Display:
      | plot([56.6910021007061;113.382004201412], [170.073006302118;170.073006302118])
      | plot([113.382004201412;170.073006302118], [85.0365031510592;85.0365031510592])
      | plot([0;226.764008402824;226.764008402824;0;0], [226.764008402824;226.764008402824;0;0;226.764008402824])
      | plot([113.382004201412;113.382004201412], [141.727505251765;198.418507352471])
      | plot([102.043803781271;124.720204621553], [198.418507352471;198.418507352471])
      | plot([102.043803781271;124.720204621553], [141.727505251765;141.727505251765])
      | plot([102.043803781271;124.720204621553], [130.389304831624;130.389304831624])
      | plot([102.043803781271;124.720204621553], [39.6837014704943;39.6837014704943])
      | plot([113.382004201412;113.382004201412], [130.389304831624;39.6837014704943])
  "Power Coupler " : Subsystem
      mask Display: image(imread('transmission.jpg'))
  Rear Gear : Subsystem
      mask Display:
      | plot([56.6910021007061;113.382004201412], [170.073006302118;170.073006302118])
      | plot([113.382004201412;170.073006302118], [85.0365031510592;85.0365031510592])
      | plot([0;226.764008402824;226.764008402824;0;0], [226.764008402824;226.764008402824;0;0;226.764008402824])
      | plot([113.382004201412;113.382004201412], [141.727505251765;198.418507352471])
      | plot([102.043803781271;124.720204621553], [198.418507352471;198.418507352471])
      | plot([102.043803781271;124.720204621553], [141.727505251765;141.727505251765])
      | plot([102.043803781271;124.720204621553], [130.389304831624;130.389304831624])
      | plot([102.043803781271;124.720204621553], [39.6837014704943;39.6837014704943])
      | plot([113.382004201412;113.382004201412], [130.389304831624;39.6837014704943])
  Simulation Results : Subsystem
      mask Display: image(imread('results.jpg'))
  Vehicle dynamics : Subsystem
      mask Display: image(imread('SUV.jpg'));
  engine : Subsystem
      mask Display: image(imread('power_HEV_powertrain_ths.jpg'))
  motorA : Subsystem
      mask Display: image(imread('power_HEV_powertrain_syncgenerator.jpg'))
  motorB : Subsystem
      mask Display: image(imread('power_HEV_powertrain_syncgenerator.jpg'))
  motorZ_default_zero : Constant  Value=0  OutDataTypeStr=double
  tag scope: PZ_com=global, PZ_ele=global, PZ_mech=global, PZ_ref=global, TZ_act=global, TZ_ref=global, nZ_act=global, nZ_ref=global, voltageZ=global
  wires:
  motorZ_default_zero/1 -> [TZ_ref], [TZ_act], [voltageZ], [PZ_ele], [PZ_mech], [nZ_act], [nZ_ref], [PZ_com], [PZ_ref]
  connections:
  Front Gear/LConn1 -- engine/RConn1
  "Power Coupler "/LConn1 -- motorA/RConn1
  motorB/LConn1 -- "Power Coupler "/RConn1
  motorB/RConn1 -- motorA/LConn1 -- Battery/LConn1
  motorB/RConn2 -- motorA/LConn2 -- Battery/LConn2
  Rear Gear/RConn1 -- Vehicle dynamics/LConn1
  Rear Gear/LConn1 -- "Power Coupler "/RConn2
  Front Gear/RConn1 -- "Power Coupler "/LConn2
